simulink model "yvle"  (R2018b)
settings: Solver=VariableStepAuto  StartTime=0.0  StopTime=5  RelTol=1e-3
settings Model: Creator=19810  LastModifiedBy=19810

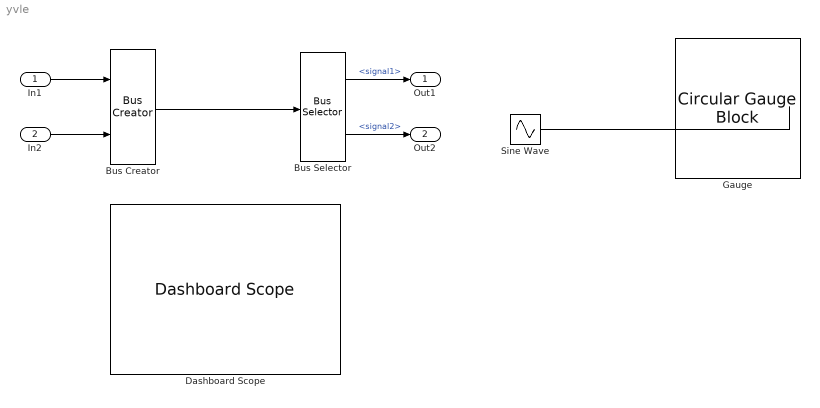
== system yvle ==
  In1 : Inport
  In2 : Inport  Port=2
  Bus Creator : BusCreator  Inputs=2
  Bus Selector : BusSelector  OutputSignals=signal1,signal2
  Dashboard Scope : DashboardScope  WebBlockId=8
  Gauge : CircularGaugeBlock  WebBlockId=9
  Sine Wave : Sin  Amplitude=100  SampleTime=0
  Out1 : Outport
  Out2 : Outport  Port=2
  wires:
  In1/1 -> Bus Creator/1
  In2/1 -> Bus Creator/2
  Bus Creator/1 -> Bus Selector/1
  Bus Selector/1 -> Out1/1  "<signal1>"
  Bus Selector/2 -> Out2/1  "<signal2>"
  Sine Wave/1 -> ?
